simulink subsystem "Driveline3W"  (R2025b)
settings: Solver=VariableStepAuto  StartTime=0.0  StopTime=10.0  RelTol=1e-3
undefined symbols (not defined in the file or in its folder): drivetrain
libraries: fl_lib x7, sdl_lib x6, nesl_utility x2
settings Model: Creator=jjha  LastModifiedBy=jjha

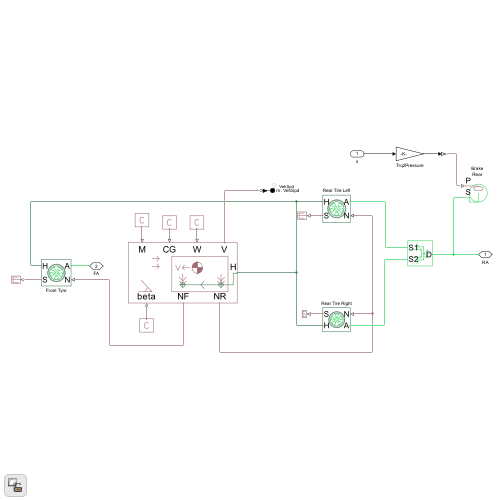
[thumbnail: Simulink's stored preview of the top-level diagram]
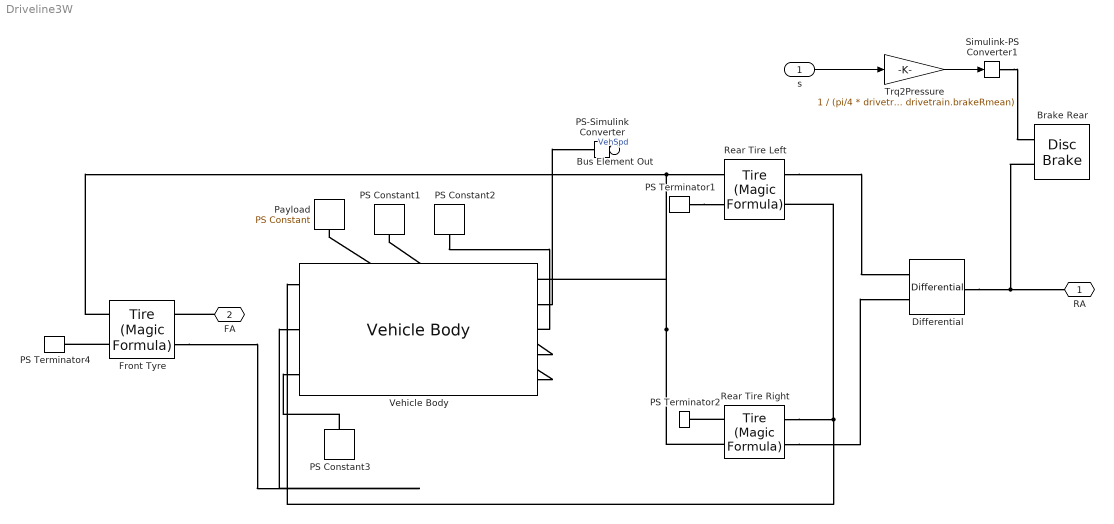
== system Driveline3W ==
  s : Inport
  Brake Rear : sdl_lib/Brakes & Detents/Rotational/Disc Brake  r_mean=drivetrain.brakeRmean m  bore=drivetrain.brakeBore m  n_pads=drivetrain.brakeNPads  thermal_port=simscape.enum.thermaleffects.omit  mu_static=drivetrain.brakeMuCoulomb * 1.2  mu_coulomb=drivetrain.brakeMuCoulomb  temperature_TLU=[280, 300, 320] K  mu_static_TLU=[.9, .8, .7]  mu_coulomb_TLU=[.8, .7, .6]  brkwy_vel=0.1 rad/s  visc_coef=0 N*m*s/rad  thermal_mass=50 kJ/K  temperature_specify=off  temperature_priority=High  temperature=300 K  temperature_nominal_specify=off  temperature_nominal_value=1  temperature_nominal_unit=K
  Differential : sdl_lib/Gears/Differential  driveshaft_location=sdl.enum.differential_orientation.right  cd_ratio=drivetrain.gearRatio  friction_model=sdl.enum.gear_friction.none  efficiency=[.85, .92]  temperature_TLU=[280, 300, 320] K  efficiency_ss_TLU=[.95, .9, .85]  efficiency_cd_TLU=[.95, .9, .85]  pwr_thr=[.001, .001] W  mu_visc=[0, 0] N*m*s/rad  model_inertia=simscape.enum.onoff.off  sun_inertia=1e-10 kg*m^2  sun_radius=0.01 m  carrier_inertia=0.001 kg*m^2  planet_inertia=0.001 kg*m^2  planet_mass=1e-10 kg  thermal_mass=50 J/K  T_init=300 K
  Front Tyre : sdl_lib/Tires & Vehicles/Tire (Magic Formula)  parameterization=sdl.enum.magic_tire_model.peak  F_z1=drivetrain.ratedVerticalLoad_N N  F_x1=drivetrain.ratedVerticalLoad_N N  kappa1=drivetrain.slipPeakForce_perc  B_m=10  C_m=1.9  D_m=1  E_m=0.97  fz0=4000 N  p_Cx=1.685  p_Dx=[1.21, -.037]  p_Ex=[.344, .095, -.02, 0]  p_Kx=[21.51, -.163, .245]  p_Hx=[-.002, .002]  p_Vx=[0, 0]  rolling_radius_model=sdl.enum.RollingRadiusParameterization.Constant  r_e=drivetrain.tireRollingRadius_m m  r_0=0.3 m  breff=8.39  dreff=0.26  freff=0.074  q_re0=0.99  q_v1=0.008  longvl=17 m/s  cz=5e5 N/m  model_resistance=true  resistance_model=sdl.enum.rollingResistanceParameterization.constant  coeff=drivetrain.rollingResistanceCoeff  p_tire=250e3 Pa  alpha=-0.003  beta=0.97  coeff_a=84e-4  coeff_b=6.2e-4 s/m  coeff_c=1.6e-4 s^2/m^2  p_tire0=240e3 Pa  fz0_resistance=4000 N  vH0=16 m/s  q_Sy=[.0082, 0, .0014, .001, 0, 0, 1.08, -.5]  v_thr=0.001 m/s  enable_scaling_coefficients=false  lfzO=1  lcx=1  lmux=1  lex=1  lkx=1  lhx=1  lvx=1  lmy=1  model_compliance=sdl.enum.compliance.off  stiffness=1e6 N/m  damping=1000 N*s/m  model_inertia=sdl.enum.model_inertia.off  inertia=1 kg*m^2  initial_velocity=0 rad/s  vxlow=1 m/s  v_tr_thr=0.1 m/s  kpumin=-1.5  kpumax=1.5
  PS Constant1 : fl_lib/Physical Signals/Sources/PS Constant  constant=drivetrain.payloadCG
  PS Constant2 : fl_lib/Physical Signals/Sources/PS Constant  constant=0
  PS Constant3 : fl_lib/Physical Signals/Sources/PS Constant  constant=0 rad
  PS Terminator1 : fl_lib/Physical Signals/Sinks/PS Terminator
  PS Terminator2 : fl_lib/Physical Signals/Sinks/PS Terminator
  PS Terminator4 : fl_lib/Physical Signals/Sinks/PS Terminator
  PS-Simulink Converter : nesl_utility/PS-Simulink Converter  PhysicalDomain=network_engine_domain  SubClassName=ps_output  LeftPortType=input  RightPortType=output  PseudoPeriodic=off  Frequencies=[]  VectorFormat=inherit  Unit=km/hr  AffineConversion=off
  Payload : fl_lib/Physical Signals/Sources/PS Constant  constant=drivetrain.payload_kg kg
  Rear Tire Left : sdl_lib/Tires & Vehicles/Tire (Magic Formula)  parameterization=sdl.enum.magic_tire_model.peak  F_z1=drivetrain.ratedVerticalLoad_N N  F_x1=drivetrain.peakLongForce_N N  kappa1=drivetrain.slipPeakForce_perc  B_m=10  C_m=1.9  D_m=1  E_m=0.97  fz0=4000 N  p_Cx=1.685  p_Dx=[1.21, -.037]  p_Ex=[.344, .095, -.02, 0]  p_Kx=[21.51, -.163, .245]  p_Hx=[-.002, .002]  p_Vx=[0, 0]  rolling_radius_model=sdl.enum.RollingRadiusParameterization.Constant  r_e=drivetrain.tireRollingRadius_m m  r_0=0.3 m  breff=8.39  dreff=0.26  freff=0.074  q_re0=0.99  q_v1=0.008  longvl=17 m/s  cz=5e5 N/m  model_resistance=true  resistance_model=sdl.enum.rollingResistanceParameterization.constant  coeff=drivetrain.rollingResistanceCoeff  p_tire=250e3 Pa  alpha=-0.003  beta=0.97  coeff_a=84e-4  coeff_b=6.2e-4 s/m  coeff_c=1.6e-4 s^2/m^2  p_tire0=240e3 Pa  fz0_resistance=4000 N  vH0=16 m/s  q_Sy=[.0082, 0, .0014, .001, 0, 0, 1.08, -.5]  v_thr=0.001 m/s  enable_scaling_coefficients=false  lfzO=1  lcx=1  lmux=1  lex=1  lkx=1  lhx=1  lvx=1  lmy=1  model_compliance=sdl.enum.compliance.off  stiffness=1e6 N/m  damping=1000 N*s/m  model_inertia=sdl.enum.model_inertia.off  inertia=1 kg*m^2  initial_velocity=0 rad/s  vxlow=1 m/s  v_tr_thr=0.1 m/s  kpumin=-1.5  kpumax=1.5
  Rear Tire Right : sdl_lib/Tires & Vehicles/Tire (Magic Formula)  parameterization=sdl.enum.magic_tire_model.peak  F_z1=drivetrain.ratedVerticalLoad_N N  F_x1=drivetrain.peakLongForce_N N  kappa1=drivetrain.slipPeakForce_perc  B_m=10  C_m=1.9  D_m=1  E_m=0.97  fz0=4000 N  p_Cx=1.685  p_Dx=[1.21, -.037]  p_Ex=[.344, .095, -.02, 0]  p_Kx=[21.51, -.163, .245]  p_Hx=[-.002, .002]  p_Vx=[0, 0]  rolling_radius_model=sdl.enum.RollingRadiusParameterization.Constant  r_e=drivetrain.tireRollingRadius_m m  r_0=0.3 m  breff=8.39  dreff=0.26  freff=0.074  q_re0=0.99  q_v1=0.008  longvl=17 m/s  cz=5e5 N/m  model_resistance=true  resistance_model=sdl.enum.rollingResistanceParameterization.constant  coeff=drivetrain.rollingResistanceCoeff  p_tire=250e3 Pa  alpha=-0.003  beta=0.97  coeff_a=84e-4  coeff_b=6.2e-4 s/m  coeff_c=1.6e-4 s^2/m^2  p_tire0=240e3 Pa  fz0_resistance=4000 N  vH0=16 m/s  q_Sy=[.0082, 0, .0014, .001, 0, 0, 1.08, -.5]  v_thr=0.001 m/s  enable_scaling_coefficients=false  lfzO=1  lcx=1  lmux=1  lex=1  lkx=1  lhx=1  lvx=1  lmy=1  model_compliance=sdl.enum.compliance.off  stiffness=1e6 N/m  damping=1000 N*s/m  model_inertia=sdl.enum.model_inertia.off  inertia=1 kg*m^2  initial_velocity=0 rad/s  vxlow=1 m/s  v_tr_thr=0.1 m/s  kpumin=-1.5  kpumax=1.5
  Simulink-PS Converter1 : nesl_utility/Simulink-PS Converter  PhysicalDomain=network_engine_domain  SubClassName=ps_input  LeftPortType=input  RightPortType=output  PseudoPeriodic=off  Frequencies=[]  NoiseDistribution=none  NoiseParameters=[]  Unit=Pa  AffineConversion=off  FilteringAndDerivatives=provide  SimscapeFilterOrder=1  InputFilterTimeConstant=0.001  UdotUserProvided=0
  Trq2Pressure : Gain  Gain=1 / (pi/4 * drivetrain.brakeBore^2 * drivetrain.brakeNPads * drivetrain.brakeMuCoulomb * drivetrain.brakeRmean)
  Vehicle Body : sdl_lib/Tires & Vehicles/Vehicle Body  mass=drivetrain.vehMass_kg kg  n_w=drivetrain.numWhlAxle  x_f=drivetrain.distCGFrontAxle_mm mm  x_r=drivetrain.distCGRearAxle_mm mm  y_c=drivetrain.cgHeight_mm mm  mass_var=true  g=drivetrain.g_mps2 m/s^2  liftoff_warning=simscape.enum.onoff.off  area=drivetrain.frontalArea_m2 m^2  Cd_var=false  Cd=drivetrain.dragCoeff  rho=drivetrain.airDensity_kgpm3 kg/m^3  model_pitch=simscape.enum.onoff.off  inertia=4000 kg*m^2  suspension_model=sdl.enum.linearTLU.linear  k_f=1e4 N/m  b_f=1e4 N*s/m  k_r=1e4 N/m  b_r=1e4 N*s/m  k_f_TLU=[-2000, -1000, 0, 1000, 2000] N  x_f_TLU=[-.4, -.2, 0, .2, .4] m  b_f_TLU=[-200, -100, 0, 100, 200] N  v_f_TLU=[-4, -2, 0, 2, 4] m/s  k_r_TLU=[-2000, -1000, 0, 1000, 2000] N  x_r_TLU=[-.4, -.2, 0, .2, .4] m  b_r_TLU=[-200, -100, 0, 100, 200] N  v_r_TLU=[-4, -2, 0, 2, 4] m/s  interp_method=simscape.enum.interpolation.linear  extrap_method=simscape.enum.extrapolation.linear  model_hardstop=simscape.enum.onoff.off  upper_bound_f=.25 m  lower_bound_f=-.25 m  stop_k_f=1e6 N/m  stop_b_f=150 N*s/m  upper_bound_r=.25 m  lower_bound_r=-.25 m  stop_k_r=1e6 N/m  stop_b_r=150 N*s/m  initial_pitch=0 rad  initial_pitch_rate=0 rad/s  v_specify=off  v_priority=High  v=25 km/hr  v_nominal_specify=off  v_nominal_value=15  v_nominal_unit=m/s
      settings: InternalSimscapePortConfiguration="{\"Bottom\":[{\"id\":\"NR\",\"label\":\"NR\",\"type\":\"output\"},{\"id\":\"NF\",\"label\":\"NF\",\"type\":\"output\"},{\"id\":\"beta\",\"label\":\"beta\",\"type\":\"input\"}],\"Left\":[{\"id\":\"H\",\"label\":\"H\",\"type\":\"foundation.mechanical.translational.translational\"}],\"Right\":[],\"Top\":[{\"id\":\"V\",\"label\":\"V\",\"type\":\"output\"},{\"id\":\"wind\",\"label\":\"W\",\"type\":\"input\"},{\"id\":\"cg_load\",\"label\":\"CG\",\"type\":\"input\"},{\"id\":\"mass_load\",\"label\":\"M\",\"type\":\"input\"}]}"
  RA : PMIOPort  Side=Left
  FA : PMIOPort  Port=2  Side=Right
  Bus Element Out : Outport  PortName=m  Element=VehSpd
  wires:
  Trq2Pressure/1 -> Simulink-PS Converter1/1
  PS-Simulink Converter/1 -> Bus Element Out/1  "VehSpd"
  s/1 -> Trq2Pressure/1
  connections:
  Rear Tire Left/LConn1 -- Rear Tire Right/LConn1 -- Vehicle Body/RConn1
  Rear Tire Right/RConn2 -- Rear Tire Left/RConn2 -- Front Tyre/RConn2 -- Vehicle Body/LConn1
  Differential/LConn1 -- Brake Rear/LConn2 -- RA/RConn1
  Vehicle Body/LConn2 -- PS-Simulink Converter/LConn1
  PS Constant2/RConn1 -- Vehicle Body/LConn3
  Vehicle Body/LConn5 -- Payload/RConn1
  PS Constant3/RConn1 -- Vehicle Body/RConn3
  Vehicle Body/LConn4 -- PS Constant1/RConn1
  Front Tyre/LConn1 -- Vehicle Body/RConn2
  Front Tyre/RConn1 -- PS Terminator4/LConn1
  FA/RConn1 -- Front Tyre/LConn2
  Rear Tire Right/RConn1 -- PS Terminator2/LConn1
  Rear Tire Left/LConn2 -- Differential/RConn1
  Rear Tire Right/LConn2 -- Differential/RConn2
  Simulink-PS Converter1/RConn1 -- Brake Rear/LConn1
  PS Terminator1/LConn1 -- Rear Tire Left/RConn1
